simulink model "half_car"  (R2021b)
settings: Solver=VariableStepAuto  StartTime=0.0  StopTime=10.0  RelTol=1e-3
settings Model: Creator=Emil Chodowiec  LastModifiedBy=Emil Chodowiec

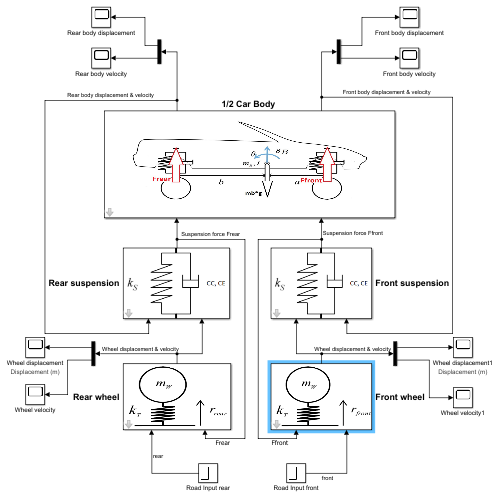
[thumbnail: Simulink's stored preview of the top-level diagram]
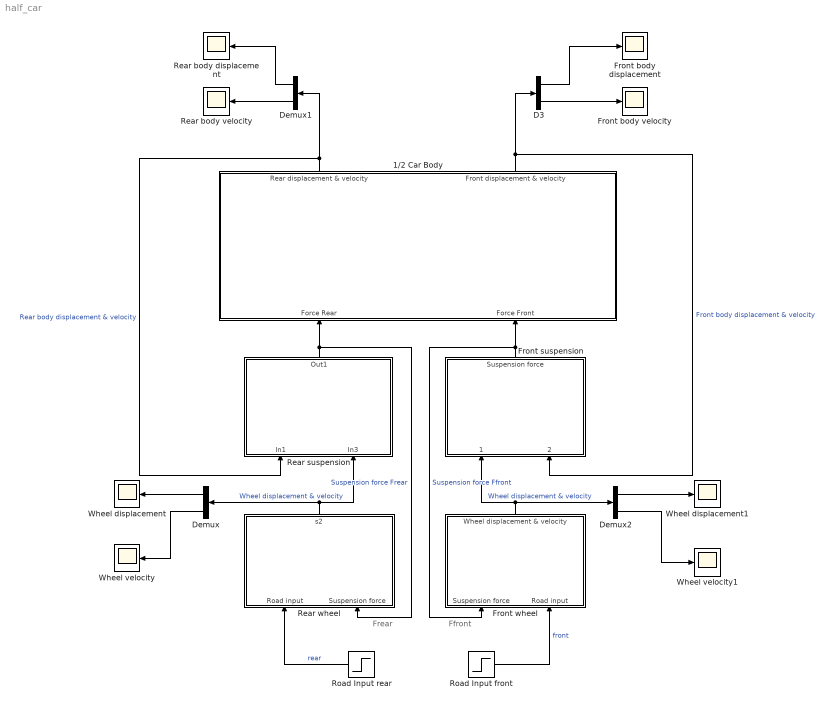
== system half_car ==
  note: Ffront
  note: Frear
  "1/2 Car Body " : Subsystem  mask{mb=500, I=600, g=9.81, a=1.25, b=1.4}
      mask prompts: mb "Body mass (mb) [kg]"; I "Inertia (I) [kg/m^2]"; g "Gravitational accelaration (g) [m/s^2]"; a "Length (a) [m]"; b "Length (b) [m]"
      settings: PortSchema="{\"entries\":[{\"content\":{\"sides\":[{\"content\":{\"connectorIds\":[]},\"type\":\"ConnectorPlacement.EquallySpacedRectSide\",\"uuid\":\"44a9b318-95d7-481a-8c99-a4baf43b2a54\"},{\"content\":{\"connectorIds\":[],\"side\":\"RIGHT\"},\"type\":\"ConnectorPlacement.EquallySpacedRectSide\",\"uuid\":\"fdd860b9-d083-49d6-8f7b-79d3eabc6cb0\"},{\"content\":{\"connectorIds\":[\"Out1\",\"Out2\"],\"side\":\"TOP\"},\"type\":\"ConnectorPlacement.EquallySpacedRectSide\",\"uuid\":\"d702ca3f-6dc3-4768-821e-f59bdd6d96df\"},{\"content\":{\"connectorIds\":[\"In1\",\"In2\"],\"side\":\"BOTTOM\"},\"type\":\"ConnectorPlacement.EquallySpacedRectSide\",\"uuid\":\"749510d2-c978-479c-910c-a4cafe277161\"}]},\"type\":\"ConnectorPlacement.EquallySpacedConnector\",\"uuid\":\"88f5b961-0f4b-41b8-b62e-bf03138c7783\"}],\"packageUris\":[\"http://schema.mathworks.com/mf0/Connector/R2020b\"],\"version\":\"1.0\"}"
      mask DialogControl DescGroupVar Prompt: 1/2 Car Body Model
      mask DialogControl DescTextVar Prompt: Please define vehicle body parameters below.
      mask Display: disp('1/2 car body')
  D3 : Demux  Outputs=2
  Demux : Demux  Outputs=2
  Demux1 : Demux  Outputs=2
  Demux2 : Demux  Outputs=2
  Front body displacement : Scope
  Front body velocity : Scope
  Front suspension : Subsystem  mask{ks=20000, cc=600, ce=1200, x0=0.2, x1=1}
      mask prompts: ks "Spring stifness (ks) [N/m]"; cc "Damping contraction (cc) [Ns/m]"; ce "Damping extension (ce) [Ns/m]"
      settings: PortSchema="{\"entries\":[{\"content\":{\"sides\":[{\"content\":{\"connectorIds\":[]},\"type\":\"ConnectorPlacement.EquallySpacedRectSide\",\"uuid\":\"c839a6a4-d4ac-4afe-8880-4c0ec4a5305a\"},{\"content\":{\"connectorIds\":[],\"side\":\"RIGHT\"},\"type\":\"ConnectorPlacement.EquallySpacedRectSide\",\"uuid\":\"2cd93a95-1277-46cc-bf35-4d3a82cc3d70\"},{\"content\":{\"connectorIds\":[\"Out1\"],\"side\":\"TOP\"},\"type\":\"ConnectorPlacement.EquallySpacedRectSide\",\"uuid\":\"fb57aeb1-7901-4d78-97df-5146f0903319\"},{\"content\":{\"connectorIds\":[\"In1\",\"In2\"],\"side\":\"BOTTOM\"},\"type\":\"ConnectorPlacement.EquallySpacedRectSide\",\"uuid\":\"eb6cdf2e-987a-45bf-8715-4ab5fca35d40\"}]},\"type\":\"ConnectorPlacement.EquallySpacedConnector\",\"uuid\":\"df63bcdf-d0bc-41ae-92df-f2ff30792501\"}],\"packageUris\":[\"http://schema.mathworks.com/mf0/Connector/R2020b\"],\"version\":\"1.0\"}"
      mask DialogControl DescGroupVar Prompt: Front suspension.
      mask DialogControl DescTextVar Prompt: Please define front suspension parameters.
      mask Display: disp('Suspension')
  Front wheel : Subsystem  mask{kt=140000, m2=20, g=9.81}
      mask prompts: kt "Tyre stiffness (kt) [N/m]"; m2 "Tyre mass (mw) [kg]"; g "Gravitational acceleration (g) [m/s^2]"
      settings: PortSchema="{\"entries\":[{\"content\":{\"sides\":[{\"content\":{\"connectorIds\":[]},\"type\":\"ConnectorPlacement.EquallySpacedRectSide\",\"uuid\":\"c839a6a4-d4ac-4afe-8880-4c0ec4a5305a\"},{\"content\":{\"connectorIds\":[],\"side\":\"RIGHT\"},\"type\":\"ConnectorPlacement.EquallySpacedRectSide\",\"uuid\":\"2cd93a95-1277-46cc-bf35-4d3a82cc3d70\"},{\"content\":{\"connectorIds\":[\"Out1\"],\"side\":\"TOP\"},\"type\":\"ConnectorPlacement.EquallySpacedRectSide\",\"uuid\":\"fb57aeb1-7901-4d78-97df-5146f0903319\"},{\"content\":{\"connectorIds\":[\"In1\",\"In2\"],\"side\":\"BOTTOM\"},\"type\":\"ConnectorPlacement.EquallySpacedRectSide\",\"uuid\":\"8951e706-8ba8-44e3-88d2-e69c5e401cd7\"}]},\"type\":\"ConnectorPlacement.EquallySpacedConnector\",\"uuid\":\"df63bcdf-d0bc-41ae-92df-f2ff30792501\"}],\"packageUris\":[\"http://schema.mathworks.com/mf0/Connector/R2020b\"],\"version\":\"1.0\"}"
      mask DialogControl DescGroupVar Prompt: Front wheel.
      mask DialogControl DescTextVar Prompt: Please define front wheel parameters.
      mask Display: disp('Wheel')
  Rear body displacement : Scope
  Rear body velocity : Scope
  Rear suspension : Subsystem  mask{ks=20000, cc=600, ce=1200, x0=0.2, x1=1}
      mask prompts: ks "Spring stifness (ks) [N/m]"; cc "Damping contraction (cc) [Ns/m]"; ce "Damping extension (ce) [Ns/m]"
      settings: PortSchema="{\"entries\":[{\"content\":{\"sides\":[{\"content\":{\"connectorIds\":[]},\"type\":\"ConnectorPlacement.EquallySpacedRectSide\",\"uuid\":\"c839a6a4-d4ac-4afe-8880-4c0ec4a5305a\"},{\"content\":{\"connectorIds\":[],\"side\":\"RIGHT\"},\"type\":\"ConnectorPlacement.EquallySpacedRectSide\",\"uuid\":\"2cd93a95-1277-46cc-bf35-4d3a82cc3d70\"},{\"content\":{\"connectorIds\":[\"Out1\"],\"side\":\"TOP\"},\"type\":\"ConnectorPlacement.EquallySpacedRectSide\",\"uuid\":\"fb57aeb1-7901-4d78-97df-5146f0903319\"},{\"content\":{\"connectorIds\":[\"In1\",\"In2\"],\"side\":\"BOTTOM\"},\"type\":\"ConnectorPlacement.EquallySpacedRectSide\",\"uuid\":\"eb6cdf2e-987a-45bf-8715-4ab5fca35d40\"}]},\"type\":\"ConnectorPlacement.EquallySpacedConnector\",\"uuid\":\"df63bcdf-d0bc-41ae-92df-f2ff30792501\"}],\"packageUris\":[\"http://schema.mathworks.com/mf0/Connector/R2020b\"],\"version\":\"1.0\"}"
      mask DialogControl DescGroupVar Prompt: Rear suspension
      mask DialogControl DescTextVar Prompt: Please define rear suspension parameters.
      mask Display: disp('Suspension')
  Rear wheel : Subsystem  mask{kt=140000, m2=20, g=9.81}
      mask prompts: kt "Tyre stiffness (kt) [N/m]"; m2 "Tyre mass (mw) [kg]"; g "Gravitational acceleration (g) [m/s^2]"
      settings: PortSchema="{\"entries\":[{\"content\":{\"sides\":[{\"content\":{\"connectorIds\":[]},\"type\":\"ConnectorPlacement.EquallySpacedRectSide\",\"uuid\":\"c839a6a4-d4ac-4afe-8880-4c0ec4a5305a\"},{\"content\":{\"connectorIds\":[],\"side\":\"RIGHT\"},\"type\":\"ConnectorPlacement.EquallySpacedRectSide\",\"uuid\":\"2cd93a95-1277-46cc-bf35-4d3a82cc3d70\"},{\"content\":{\"connectorIds\":[\"Out1\"],\"side\":\"TOP\"},\"type\":\"ConnectorPlacement.EquallySpacedRectSide\",\"uuid\":\"fb57aeb1-7901-4d78-97df-5146f0903319\"},{\"content\":{\"connectorIds\":[\"In1\",\"In2\"],\"side\":\"BOTTOM\"},\"type\":\"ConnectorPlacement.EquallySpacedRectSide\",\"uuid\":\"8951e706-8ba8-44e3-88d2-e69c5e401cd7\"}]},\"type\":\"ConnectorPlacement.EquallySpacedConnector\",\"uuid\":\"df63bcdf-d0bc-41ae-92df-f2ff30792501\"}],\"packageUris\":[\"http://schema.mathworks.com/mf0/Connector/R2020b\"],\"version\":\"1.0\"}"
      mask DialogControl DescGroupVar Prompt: Rear wheel.
      mask DialogControl DescTextVar Prompt: Please define rear wheel parameters.
      mask Display: disp('Wheel')
  Road Input front : Step  After=0  SampleTime=0
  Road Input rear : Step  After=0  SampleTime=0
  Wheel displacement : Scope
      settings: AttributesFormatString=%<YLabel>
  Wheel displacement1 : Scope
      settings: AttributesFormatString=%<YLabel>
  Wheel velocity : Scope
  Wheel velocity1 : Scope
  wires:
  Road Input front/1 -> Front wheel/2(Road input)  "front"
  "1/2 Car Body "/1(Rear displacement & velocity) -> Demux1/1, Rear suspension/1(In1)  "Rear body displacement & velocity"
  Road Input rear/1 -> Rear wheel/1(Road input)  "rear"
  Demux2/2 -> Wheel velocity1/1
  Front wheel/1(Wheel displacement & velocity) -> Front suspension/1(Wheel displacement & velocity), Demux2/1  "Wheel displacement & velocity"
  Demux1/1 -> Rear body displacement/1
  "1/2 Car Body "/2(Front displacement & velocity) -> D3/1, Front suspension/2(Body displacement & velocity)  "Front body displacement & velocity"
  Rear wheel/1(s2) -> Rear suspension/2(In3), Demux/1  "Wheel displacement & velocity"
  D3/2 -> Front body velocity/1
  Demux2/1 -> Wheel displacement1/1
  Front suspension/1(Suspension force) -> "1/2 Car Body "/2(Force Front), Front wheel/1(Suspension force)  "Suspension force Ffront"
  D3/1 -> Front body displacement/1
  Rear suspension/1(Out1) -> "1/2 Car Body "/1("Force Rear "), Rear wheel/2(Suspension force)  "Suspension force Frear"
  Demux/2 -> Wheel velocity/1
  Demux/1 -> Wheel displacement/1
  Demux1/2 -> Rear body velocity/1

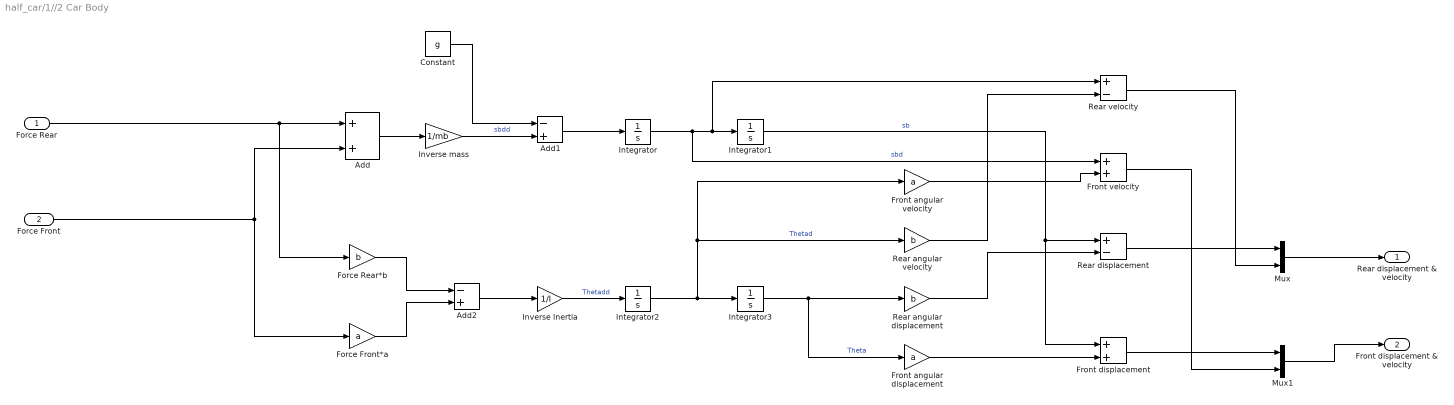
== system half_car/1//2 Car Body  ==
  "Force Rear " : Inport
  Force Front : Inport  Port=2
  Add : Sum
  Add1 : Sum  Inputs=-+
  Add2 : Sum  Inputs=-+
  Constant : Constant  Value=g
  Force Front*a : Gain  Gain=a
  Force Rear*b : Gain  Gain=b
  Front angular displacement : Gain  Gain=a
  Front angular velocity : Gain  Gain=a
  Front displacement : Sum
  Front velocity : Sum
  Integrator{,1..3} (4 alike) : Integrator
  Inverse Inertia : Gain  Gain=1/I
  Inverse mass : Gain  Gain=1/mb
  Mux : Mux  Inputs=2
  Mux1 : Mux  Inputs=2
  Rear angular displacement : Gain  Gain=b
  Rear angular velocity : Gain  Gain=b
  Rear displacement : Sum  Inputs=+-
  Rear velocity : Sum  Inputs=+-
  Rear displacement & velocity : Outport
  Front displacement & velocity : Outport  Port=2
  wires:
  Force Front/1 -> Add/2, Force Front*a/1
  Add/1 -> Inverse mass/1
  Integrator/1 -> Front velocity/1, Rear velocity/1, Integrator1/1  "sbd"
  Constant/1 -> Add1/1
  Inverse mass/1 -> Add1/2  "sbdd"
  Add1/1 -> Integrator/1
  Integrator1/1 -> Front displacement/1, Rear displacement/1  "sb"
  Force Front*a/1 -> Add2/2
  Force Rear*b/1 -> Add2/1
  Add2/1 -> Inverse Inertia/1
  Inverse Inertia/1 -> Integrator2/1  "Thetadd"
  Integrator2/1 -> Front angular velocity/1, Rear angular velocity/1, Integrator3/1  "Thetad"
  Integrator3/1 -> Front angular displacement/1, Rear angular displacement/1  "Theta"
  "Force Rear "/1 -> Force Rear*b/1, Add/1
  Rear angular displacement/1 -> Rear displacement/2
  Front angular displacement/1 -> Front displacement/2
  Mux/1 -> Rear displacement & velocity/1
  Mux1/1 -> Front displacement & velocity/1
  Front velocity/1 -> Mux1/2
  Rear displacement/1 -> Mux/1
  Front displacement/1 -> Mux1/1
  Rear velocity/1 -> Mux/2
  Rear angular velocity/1 -> Rear velocity/2
  Front angular velocity/1 -> Front velocity/2

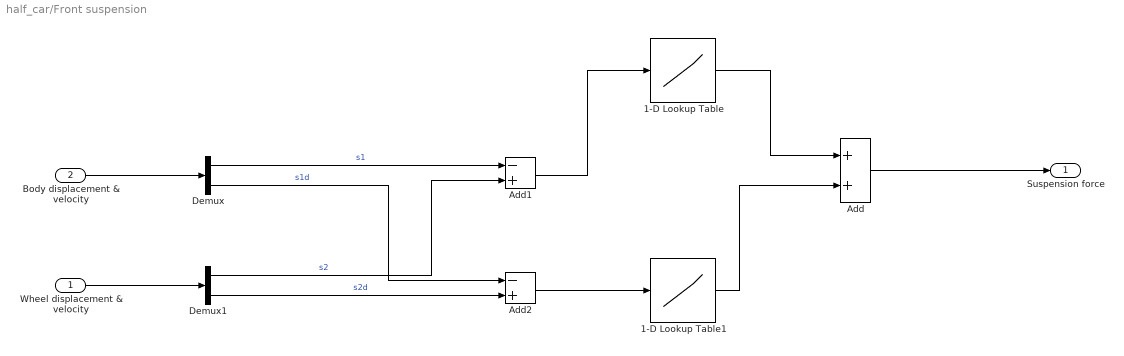
== system half_car/Front suspension ==
  Wheel displacement & velocity : Inport
  Body displacement & velocity : Inport  Port=2
  1-D Lookup Table : Lookup_n-D  NumberOfTableDimensions=1  BreakpointsForDimension1=[-2*x0, -x0, x0, 2*x0]  Table=[-(ks+20*ks)*x0, -ks*x0, ks*x0, (ks+ks*20)*x0]  InternalRulePriority=Speed  RndMeth=Simplest  InputSameDT=on
  1-D Lookup Table1 : Lookup_n-D  NumberOfTableDimensions=1  BreakpointsForDimension1=[-x1, 0, x1]  Table=[-ce*x1, 0, cc*x1]  InternalRulePriority=Speed  RndMeth=Simplest  InputSameDT=on
  Add : Sum
  Add1 : Sum  Inputs=-+
  Add2 : Sum  Inputs=-+
  Demux : Demux  Outputs=2
  Demux1 : Demux  Outputs=2
  Suspension force : Outport
  wires:
  1-D Lookup Table/1 -> Add/1
  Add/1 -> Suspension force/1
  Demux/1 -> Add1/1  "s1"
  Add1/1 -> 1-D Lookup Table/1
  Demux/2 -> Add2/1  "s1d"
  Body displacement & velocity/1 -> Demux/1
  Wheel displacement & velocity/1 -> Demux1/1
  Demux1/1 -> Add1/2  "s2"
  Demux1/2 -> Add2/2  "s2d"
  Add2/1 -> 1-D Lookup Table1/1
  1-D Lookup Table1/1 -> Add/2

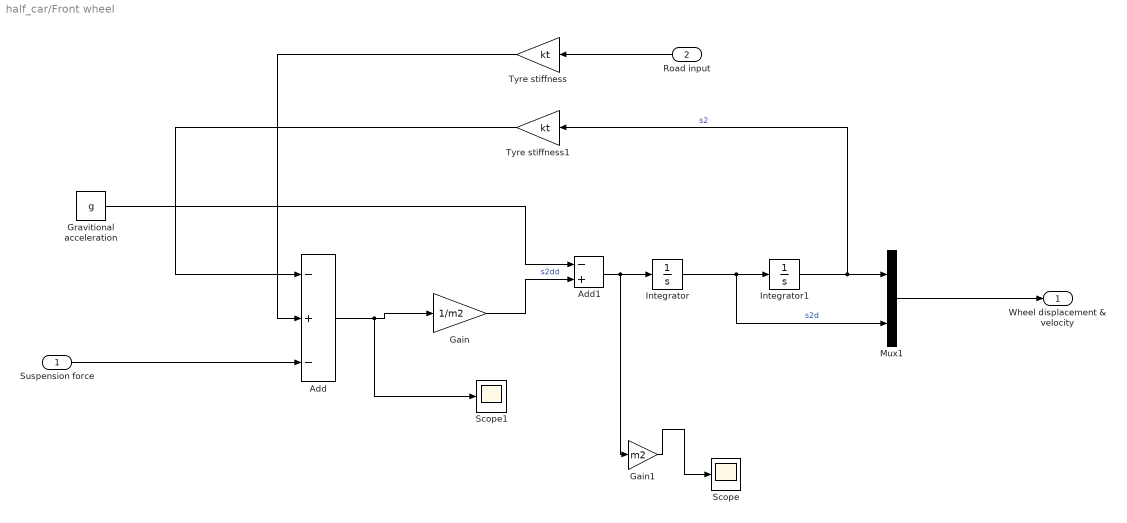
== system half_car/Front wheel ==
  Suspension force : Inport
  Road input : Inport  Port=2
  Add : Sum  Inputs=-+-
  Add1 : Sum  Inputs=-+
  Gain : Gain  Gain=1/m2
  Gain1 : Gain  Gain=m2
  Gravitional acceleration : Constant  Value=g
  Integrator : Integrator
  Integrator1 : Integrator
  Mux1 : Mux  Inputs=2
  Scope : Scope
  Scope1 : Scope
  Tyre stiffness : Gain  Gain=kt
  Tyre stiffness1 : Gain  Gain=kt
  Wheel displacement & velocity : Outport
  wires:
  Integrator/1 -> Mux1/2, Integrator1/1  "s2d"
  Gravitional acceleration/1 -> Add1/1
  Add/1 -> Scope1/1, Gain/1
  Tyre stiffness/1 -> Add/2
  Tyre stiffness1/1 -> Add/1
  Integrator1/1 -> Tyre stiffness1/1, Mux1/1  "s2"
  Road input/1 -> Tyre stiffness/1
  Mux1/1 -> Wheel displacement & velocity/1
  Gain/1 -> Add1/2  "s2dd"
  Suspension force/1 -> Add/3
  Add1/1 -> Gain1/1, Integrator/1
  Gain1/1 -> Scope/1

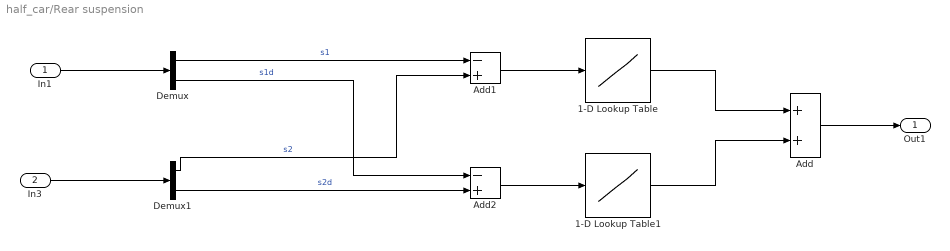
== system half_car/Rear suspension ==
  In1 : Inport
  In3 : Inport  Port=2
  1-D Lookup Table : Lookup_n-D  NumberOfTableDimensions=1  BreakpointsForDimension1=[-2*x0, -x0, x0, 2*x0]  Table=[-(ks+20*ks)*x0, -ks*x0, ks*x0, (ks+ks*20)*x0]  InternalRulePriority=Speed  RndMeth=Simplest  InputSameDT=on
  1-D Lookup Table1 : Lookup_n-D  NumberOfTableDimensions=1  BreakpointsForDimension1=[-x1, 0, x1]  Table=[-ce*x1, 0, cc*x1]  InternalRulePriority=Speed  RndMeth=Simplest  InputSameDT=on
  Add : Sum
  Add1 : Sum  Inputs=-+
  Add2 : Sum  Inputs=-+
  Demux : Demux  Outputs=2
  Demux1 : Demux  Outputs=2
  Out1 : Outport
  wires:
  1-D Lookup Table/1 -> Add/1
  Add/1 -> Out1/1
  Demux/1 -> Add1/1  "s1"
  Add1/1 -> 1-D Lookup Table/1
  Demux/2 -> Add2/1  "s1d"
  In1/1 -> Demux/1
  In3/1 -> Demux1/1
  Demux1/1 -> Add1/2  "s2"
  Demux1/2 -> Add2/2  "s2d"
  Add2/1 -> 1-D Lookup Table1/1
  1-D Lookup Table1/1 -> Add/2

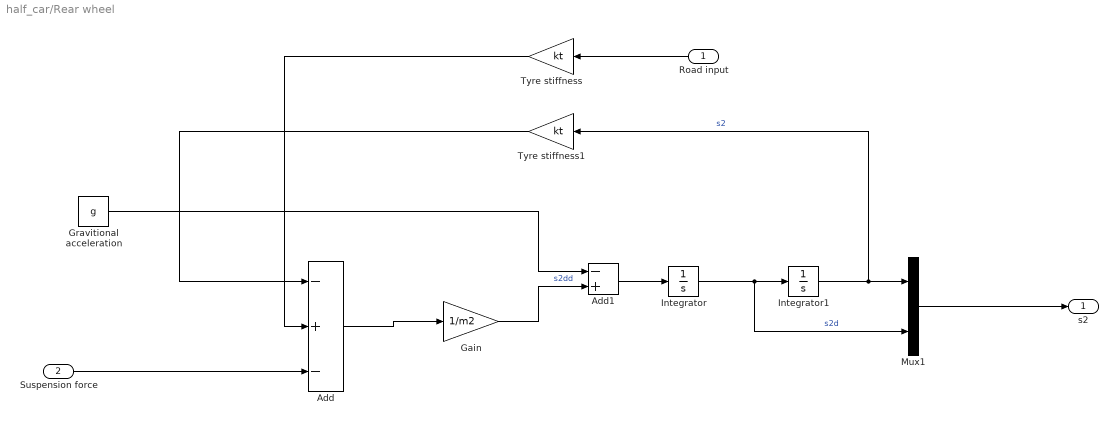
== system half_car/Rear wheel ==
  Road input : Inport
  Suspension force : Inport  Port=2
  Add : Sum  Inputs=-+-
  Add1 : Sum  Inputs=-+
  Gain : Gain  Gain=1/m2
  Gravitional acceleration : Constant  Value=g
  Integrator : Integrator
  Integrator1 : Integrator
  Mux1 : Mux  Inputs=2
  Tyre stiffness : Gain  Gain=kt
  Tyre stiffness1 : Gain  Gain=kt
  s2 : Outport
  wires:
  Integrator/1 -> Mux1/2, Integrator1/1  "s2d"
  Gravitional acceleration/1 -> Add1/1
  Add/1 -> Gain/1
  Tyre stiffness/1 -> Add/2
  Tyre stiffness1/1 -> Add/1
  Integrator1/1 -> Tyre stiffness1/1, Mux1/1  "s2"
  Road input/1 -> Tyre stiffness/1
  Mux1/1 -> s2/1
  Gain/1 -> Add1/2  "s2dd"
  Add1/1 -> Integrator/1
  Suspension force/1 -> Add/3
